simulink model "yaw_simulink1"  (R2023a)
settings: Solver=VariableStepAuto  StartTime=0.0  StopTime=10.0  RelTol=1e-3
settings Model: Creator=zhangr365  LastModifiedBy=zhangr365

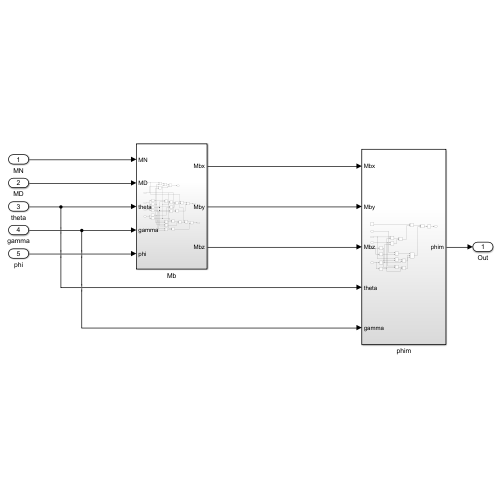
[thumbnail: Simulink's stored preview of the top-level diagram]
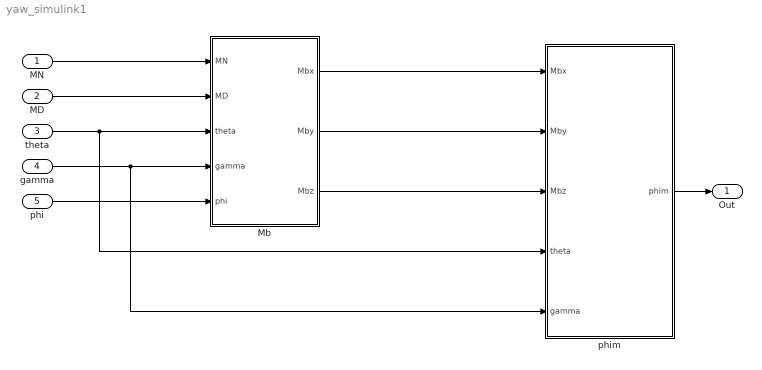
== system yaw_simulink1 ==
  MN : Inport
  MD : Inport  Port=2
  theta : Inport  Port=3
  gamma : Inport  Port=4
  phi : Inport  Port=5
  Mb : Subsystem
  phim : Subsystem
  Out : Outport
  wires:
  MN/1 -> Mb/1(MN)
  MD/1 -> Mb/2(MD)
  theta/1 -> phim/4(theta), Mb/3(theta)
  gamma/1 -> phim/5(gamma), Mb/4(gamma)
  phi/1 -> Mb/5(phi)
  Mb/1(Mbx) -> phim/1(Mbx)
  Mb/2(Mby) -> phim/2(Mby)
  Mb/3(Mbz) -> phim/3(Mbz)
  phim/1(phim) -> Out/1

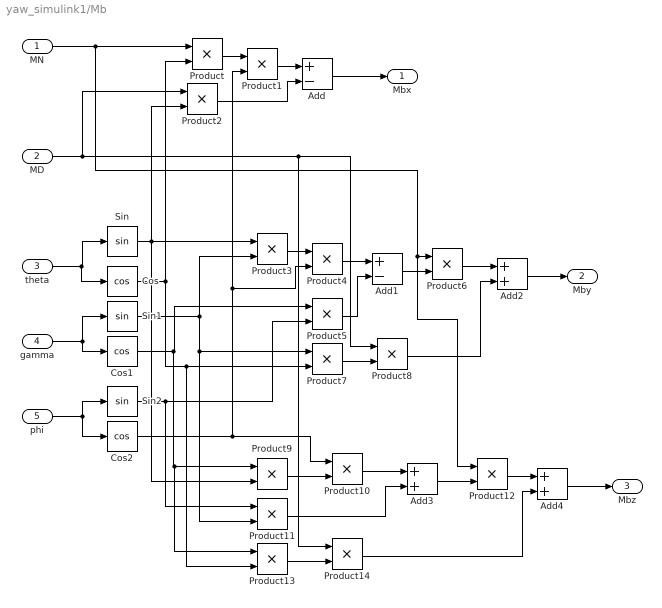
== system yaw_simulink1/Mb ==
  MN : Inport
  MD : Inport  Port=2
  theta : Inport  Port=3
  gamma : Inport  Port=4
  phi : Inport  Port=5
  Add : Sum  Inputs=+-
  Add1 : Sum  Inputs=+-
  Add2 : Sum
  Add3 : Sum
  Add4 : Sum
  Cos : Trigonometry  Operator=cos
  Cos1 : Trigonometry  Operator=cos
  Cos2 : Trigonometry  Operator=cos
  Product{,1..14} (15 alike) : Product
  Sin : Trigonometry
  Sin1 : Trigonometry
  Sin2 : Trigonometry
  Mbx : Outport
  Mby : Outport  Port=2
  Mbz : Outport  Port=3
  wires:
  Cos/1 -> Product13/2, Product7/2, Product/2
  gamma/1 -> Sin1/1, Cos1/1
  Product11/1 -> Add3/2
  Product4/1 -> Add1/1
  Add/1 -> Mbx/1
  Sin1/1 -> Product11/2, Product7/1, Product3/2
  Cos1/1 -> Product13/1, Product9/1, Product5/1
  Product12/1 -> Add4/1
  Product13/1 -> Product14/2
  Cos2/1 -> Product10/1, Product1/2, Product4/2
  Sin/1 -> Product9/2, Product2/2, Product3/1
  Add4/1 -> Mbz/1
  Add2/1 -> Mby/1
  theta/1 -> Cos/1, Sin/1
  MD/1 -> Product8/1, Product14/1, Product2/1
  Product9/1 -> Product10/2
  Product5/1 -> Add1/2
  Sin2/1 -> Product11/1, Product5/2
  Product3/1 -> Product4/1
  MN/1 -> Product12/1, Product6/1, Product/1
  Product8/1 -> Add2/2
  Add1/1 -> Product6/2
  Product6/1 -> Add2/1
  Product/1 -> Product1/1
  phi/1 -> Cos2/1, Sin2/1
  Add3/1 -> Product12/2
  Product7/1 -> Product8/2
  Product14/1 -> Add4/2
  Product2/1 -> Add/2
  Product10/1 -> Add3/1
  Product1/1 -> Add/1

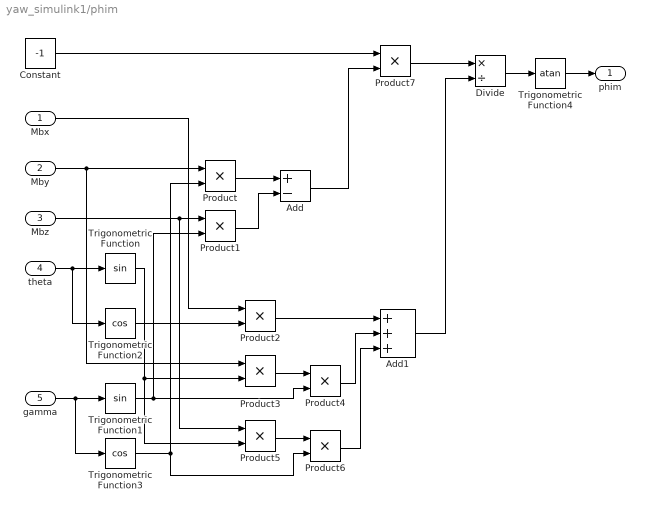
== system yaw_simulink1/phim ==
  Mbx : Inport
  Mby : Inport  Port=2
  Mbz : Inport  Port=3
  theta : Inport  Port=4
  gamma : Inport  Port=5
  Add : Sum  Inputs=+-
  Add1 : Sum  Inputs=+++
  Constant : Constant  Value=-1
  Divide : Product  Inputs=*/
  Product{,1..7} (8 alike) : Product
  Trigonometric Function : Trigonometry
  Trigonometric Function1 : Trigonometry
  Trigonometric Function2 : Trigonometry  Operator=cos
  Trigonometric Function3 : Trigonometry  Operator=cos
  Trigonometric Function4 : Trigonometry  Operator=atan
  phim : Outport
  wires:
  theta/1 -> Trigonometric Function2/1, Trigonometric Function/1
  gamma/1 -> Trigonometric Function3/1, Trigonometric Function1/1
  Mby/1 -> Product3/1, Product/1
  Trigonometric Function3/1 -> Product6/2, Product/2
  Product/1 -> Add/1
  Mbz/1 -> Product1/1, Product5/1
  Trigonometric Function1/1 -> Product4/2, Product1/2
  Product1/1 -> Add/2
  Mbx/1 -> Product2/1
  Trigonometric Function2/1 -> Product2/2
  Trigonometric Function/1 -> Product3/2, Product5/2
  Product3/1 -> Product4/1
  Product5/1 -> Product6/1
  Product2/1 -> Add1/1
  Product4/1 -> Add1/2
  Product6/1 -> Add1/3
  Constant/1 -> Product7/1
  Add/1 -> Product7/2
  Product7/1 -> Divide/1
  Add1/1 -> Divide/2
  Divide/1 -> Trigonometric Function4/1
  Trigonometric Function4/1 -> phim/1
